simulink model "Simulink_vehicle_model"  (R2024b)
settings: Solver=VariableStepAuto  StartTime=0.0  StopTime=10.0  RelTol=1e-3
libraries: autolibshared x1, mpclib x1
settings SolverCC: AlgebraicLoopSolver=TrustRegion
settings RTWCC: GPUComputeCapability=3.5

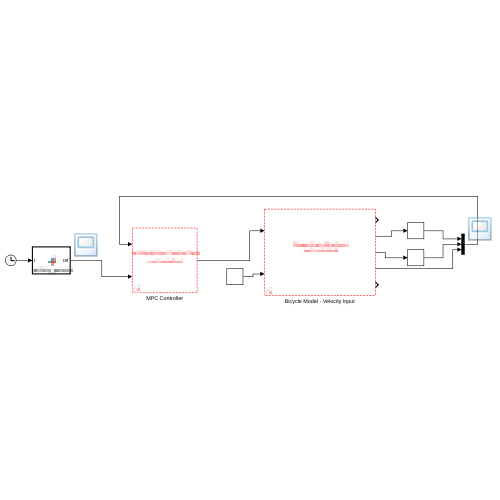
[thumbnail: Simulink's stored preview of the top-level diagram]
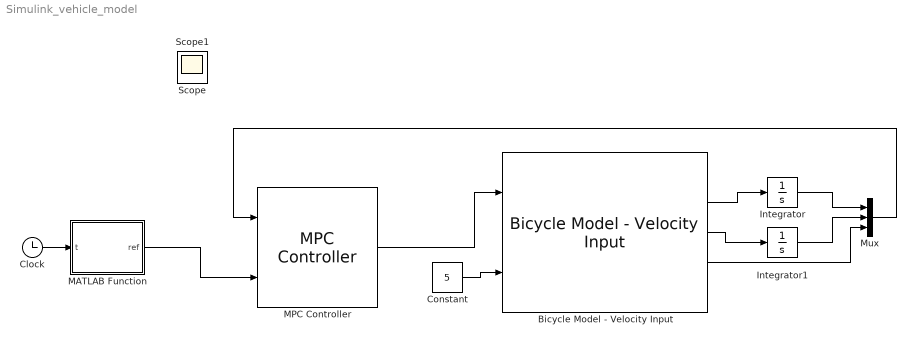
== system Simulink_vehicle_model ==
  Bicycle Model - Velocity Input : autolibshared/Bicycle Model - Velocity Input  trackMode=Single (bicycle)  inputMode=External longitudinal velocity  frontSteerMode=on  rearSteerMode=off  windMode=off  muMode=off  extFMode=off  extMMode=off  aMode=3  NF=2  NR=2  m=2000  a=1.4  b=1.6  h=0.35  X_o=0  xdot_o=0  CalphaMode=off  sigmaMode=on  w=[1.4,1.4]  Cy_f=12e3  Cy_r=11e3  sigma_f=.1  sigma_r=.1  alpha_f_brk=[-.1 .1]  Cy_f_data=[-9e3 9e3]  alpha_r_brk=[-.1 .1]  Cy_r_data=[-9e3 9e3]  Y_o=0  ydot_o=0  Izz=4000  psi_o=0  r_o=0  Af=2  Cd=.3  Cl=.1  Cpm=.1  beta_w=[0 0.01:0.01:0.3]  Cs=[0 0.01:0.01:0.3]  Cym=[0 1e-6:0.01:0.3]  Pabs=101325  Tair=273  g=9.81  mu=1  xdot_tol=.01  Fznom=5000  Fxtire_sat=1e6  Fytire_sat=1e6  longOff=0  latOff=0  vertOff=0
  Clock : Clock
  Constant : Constant  Value=5
  Integrator : Integrator
  Integrator1 : Integrator
  MATLAB Function : MATLAB Function  TreatAsAtomicUnit=on
  MPC Controller : mpclib/MPC Controller  SCDEnableBlockLinearizationSpecification=on  mpcobj=mpcController  is_multiple=0  enable_value=0  return_u0=off  updateMPCinCallerWorkspace=on  md_inport=off  mv_inport=off  uref_inport=off  return_cost=off  return_mvseq=off  return_qpstatus=off  return_xseq=off  return_state=off  return_ovseq=off  state_inport=off  umin_inport=off  umax_inport=off  ymin_inport=off  ymax_inport=off  cc_inport=off  ywt_inport=off  uwt_inport=off  duwt_inport=off  rhoeps_inport=off  pm_inport=off  MaximumP=10  HorizonChoice=FixedHorizon  n_ts=0.1  n_p=10  n_mv=1  n_md=0  n_ud=0  n_mo=3  n_uo=0  BlockDataType=double  SampleTimeInherited=off  switch_inport=off
  Mux : Mux  Inputs=3
  Scope : Scope
  Scope1 : Scope
  wires:
  MPC Controller/1 -> Bicycle Model - Velocity Input/1
  Bicycle Model - Velocity Input/2 -> Integrator/1
  Bicycle Model - Velocity Input/3 -> Integrator1/1
  Integrator/1 -> Mux/1
  Integrator1/1 -> Mux/2
  Bicycle Model - Velocity Input/4 -> Mux/3
  Mux/1 -> MPC Controller/1
  MATLAB Function/1(ref) -> MPC Controller/2
  Clock/1 -> MATLAB Function/1(t)
  Constant/1 -> Bicycle Model - Velocity Input/2

== matlab function Simulink_vehicle_model/MATLAB Function ==
  data: t input; ref output
function ref  = trajectory_generator(t)
    % Coefficients for x (e.g., 2nd-degree polynomial for x-position)
    a_x = 1; 
    b_x = 0.5; 
    c_x = 0; 
    
    % Coefficients for y (e.g., 2nd-degree polynomial for y-position)
    a_y = 1; 
    b_y = -0.3; 
    c_y = 0.2; 

    % Position equations: Polynomial trajectories
    x_pos = a_x*t^2 + b_x*t + c_x;  % x-position
    y_pos = a_y*t^2 + b_y*t + c_y;  % y-position

    % Velocity is the derivative of position
    x_vel = 2*a_x*t + b_x;  % x-velocity
    y_vel = 2*a_y*t + b_y; % y-velocity
    vel = sqrt(x_vel^2+y_vel^2);

    ref = [x_pos; y_pos; vel];
end
